simulink model "Long_Simul_1"  (R2022b)
settings: Solver=VariableStepAuto  StartTime=0.0  StopTime=Inf  RelTol=1e-3
values from neighbouring files (symbols this model uses):
  Af = 4    [Long_Simul_1_Initialize.m]    (also in Long_Simul_2_Initialize.m; Long_Simul_3_Initialize.m)
  Brake_Input_Amplitude = 100    [Long_Simul_1_Initialize.m]    (also in Long_Simul_2_Initialize.m = 10; Long_Simul_3_Initialize.m = 10)
  Brake_Input_start_time = 8    [Long_Simul_1_Initialize.m]    (also in Long_Simul_2_Initialize.m; Long_Simul_3_Initialize.m)
  C_long = 6*10^4    (= 60000)    [Long_Simul_1_Initialize.m]
  Cd = 0.3    [Long_Simul_1_Initialize.m]    (also in Long_Simul_2_Initialize.m; Long_Simul_3_Initialize.m)
  g = 9.81    [Long_Simul_1_Initialize.m]    (also in Long_Simul_2_Initialize.m; Long_Simul_3_Initialize.m)
  I_wheel = 0.8    [Long_Simul_1_Initialize.m]    (also in Long_Simul_2_Initialize.m; Long_Simul_3_Initialize.m)
  m = 1500    [Long_Simul_1_Initialize.m]    (also in Long_Simul_2_Initialize.m; Long_Simul_3_Initialize.m)
  r_eff = rw * sin(phi)/phi    [Long_Simul_1_Initialize.m]    (also in Long_Simul_2_Initialize.m; Long_Simul_3_Initialize.m)
  R_roll = 0.015    [Long_Simul_1_Initialize.m]    (also in Long_Simul_2_Initialize.m)
  rho = 1.225    [Long_Simul_1_Initialize.m]    (also in Long_Simul_2_Initialize.m; Long_Simul_3_Initialize.m)
  Throttle_Input_Amplitude = 30    [Long_Simul_1_Initialize.m]    (also in Long_Simul_2_Initialize.m; Long_Simul_3_Initialize.m = 50)
  Throttle_Input_period = 4    [Long_Simul_1_Initialize.m]    (also in Long_Simul_2_Initialize.m; Long_Simul_3_Initialize.m)
settings Model: Creator=lego0  LastModifiedBy=lego0

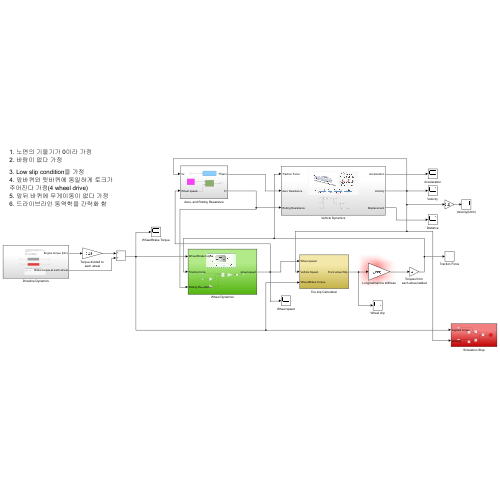
[thumbnail: Simulink's stored preview of the top-level diagram]
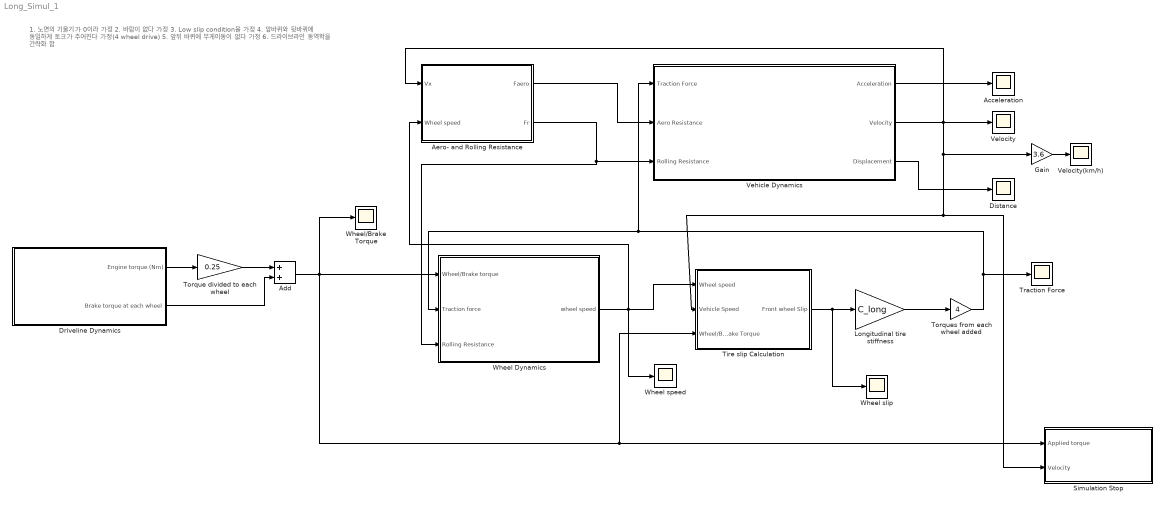
== system Long_Simul_1 ==
  note: 1. 노면의 기울기가 0이라 가정
      | 2. 바람이 없다 가정
      |
      | 3. Low slip condition을 가정
      | 4. 앞바퀴와 뒷바퀴에 동일하게 토크가 주어진다 가정(4 wheel drive)
      | 5. 앞뒤 바퀴에 무게이동이 없다 가정
      | 6. 드라이브라인 동역학을 간략화 함
  Acceleration : Scope
  Add : Sum
  Aero- and Rolling Resistance : Subsystem
  Distance : Scope
  Driveline Dynamics : Subsystem
  Gain : Gain  Gain=3.6
  Longitudinal tire stiffness : Gain  Gain=C_long
  Simulation Stop : Subsystem
  Tire slip Calculation : Subsystem
  Torque divided to each wheel : Gain  Gain=0.25
  Torques from each wheel added : Gain  Gain=4
  Traction Force : Scope
  Vehicle Dynamics : Subsystem
  Velocity : Scope
  Velocity(km/h) : Scope
  Wheel Dynamics : Subsystem
  Wheel slip : Scope
  Wheel speed : Scope
  Wheel/Brake Torque : Scope
  wires:
  Wheel Dynamics/1(wheel speed) -> Wheel speed/1, Aero- and Rolling Resistance/2(Wheel speed), Tire slip Calculation/1(Wheel speed)
  Tire slip Calculation/1(Front wheel Slip) -> Wheel slip/1, Longitudinal tire stiffness/1
  Longitudinal tire stiffness/1 -> Torques from each wheel added/1
  Vehicle Dynamics/1(Acceleration) -> Acceleration/1
  Vehicle Dynamics/2(Velocity) -> Tire slip Calculation/2(Vehicle Speed), Simulation Stop/2(Velocity), Gain/1, Velocity/1, Aero- and Rolling Resistance/1(Vx)
  Vehicle Dynamics/3(Displacement) -> Distance/1
  Gain/1 -> Velocity(km/h)/1
  Driveline Dynamics/2(Brake torque at each wheel) -> Add/2
  Aero- and Rolling Resistance/2(Fr) -> Wheel Dynamics/3(Rolling Resistance), Vehicle Dynamics/3(Rolling Resistance)
  Aero- and Rolling Resistance/1(Faero) -> Vehicle Dynamics/2(Aero Resistance)
  Add/1 -> Wheel Dynamics/1(Wheel/Brake torque), Tire slip Calculation/3(Wheel/Brake Torque), Simulation Stop/1(Applied torque), Wheel/Brake Torque/1
  Torques from each wheel added/1 -> Vehicle Dynamics/1(Traction Force), Wheel Dynamics/2(Traction force), Traction Force/1
  Driveline Dynamics/1(Engine torque (Nm)) -> Torque divided to each wheel/1
  Torque divided to each wheel/1 -> Add/1

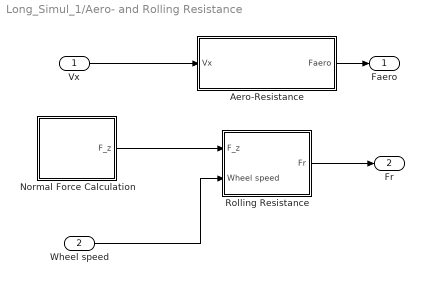
== system Long_Simul_1/Aero- and Rolling Resistance ==
  Vx : Inport
  Wheel speed : Inport  Port=2
  Aero-Resistance : Subsystem
  Normal Force Calculation : Subsystem
  Rolling Resistance : Subsystem
  Faero : Outport
  Fr : Outport  Port=2
  wires:
  Rolling Resistance/1(Fr) -> Fr/1
  Normal Force Calculation/1(F_z) -> Rolling Resistance/1(F_z)
  Vx/1 -> Aero-Resistance/1(Vx)
  Wheel speed/1 -> Rolling Resistance/2(Wheel speed)
  Aero-Resistance/1(Faero) -> Faero/1

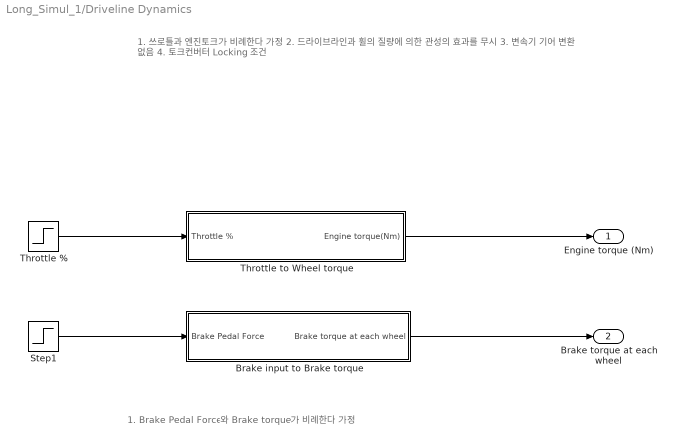
== system Long_Simul_1/Driveline Dynamics ==
  note: 1. 쓰로틀과 엔진토크가 비례한다 가정
      | 2. 드라이브라인과 휠의 질량에 의한 관성의 효과를 무시
      | 3. 변속기 기어 변환 없음
      | 4. 토크컨버터 Locking 조건
  note: 1. Brake Pedal Force와 Brake torque가 비례한다 가정
  Brake input to Brake torque : Subsystem
  Step1 : Step  Time=Brake_Input_start_time  After=Brake_Input_Amplitude  SampleTime=0
  Throttle % : Step  Time=Throttle_Input_period  Before=Throttle_Input_Amplitude  After=0  SampleTime=0
  Throttle to Wheel torque : Subsystem
  Engine torque (Nm) : Outport
  Brake torque at each wheel : Outport  Port=2
  wires:
  Throttle to Wheel torque/1(Engine torque(Nm)) -> Engine torque (Nm)/1
  Step1/1 -> Brake input to Brake torque/1(Brake Pedal Force)
  Throttle %/1 -> Throttle to Wheel torque/1(Throttle %)
  Brake input to Brake torque/1(Brake torque at each wheel) -> Brake torque at each wheel/1

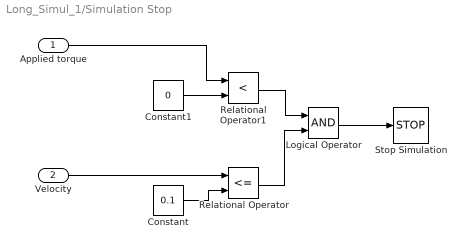
== system Long_Simul_1/Simulation Stop ==
  Applied torque : Inport
  Velocity : Inport  Port=2
  Constant : Constant  Value=0.1
  Constant1 : Constant  Value=0
  Logical Operator : Logic  AllPortsSameDT=off  OutDataTypeStr=boolean
  Relational Operator : RelationalOperator  Operator=<=  OutDataTypeStr=boolean  RndMeth=Simplest  InputSameDT=off
  Relational Operator1 : RelationalOperator  Operator=<  OutDataTypeStr=boolean  RndMeth=Simplest  InputSameDT=off
  Stop Simulation : Stop
  wires:
  Relational Operator1/1 -> Logical Operator/1
  Relational Operator/1 -> Logical Operator/2
  Constant/1 -> Relational Operator/2
  Constant1/1 -> Relational Operator1/2
  Logical Operator/1 -> Stop Simulation/1
  Velocity/1 -> Relational Operator/1
  Applied torque/1 -> Relational Operator1/1

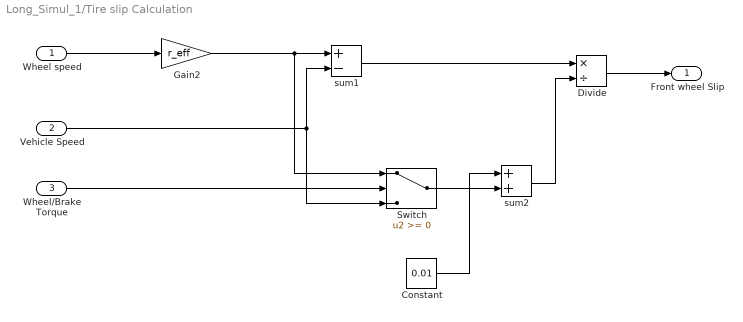
== system Long_Simul_1/Tire slip Calculation ==
  Wheel speed : Inport
  Vehicle Speed : Inport  Port=2
  Wheel/Brake Torque : Inport  Port=3
  Constant : Constant  Value=0.01
  Divide : Product  Inputs=*/
  Gain2 : Gain  Gain=r_eff
  Switch : Switch  SaturateOnIntegerOverflow=off  InputSameDT=off
  sum1 : Sum  Inputs=+-
  sum2 : Sum
  Front wheel Slip : Outport  VectorParamsAs1DForOutWhenUnconnected=off
  wires:
  Vehicle Speed/1 -> sum1/2, Switch/3
  Gain2/1 -> Switch/1, sum1/1
  Wheel speed/1 -> Gain2/1
  sum1/1 -> Divide/1
  Divide/1 -> Front wheel Slip/1
  Switch/1 -> sum2/2
  sum2/1 -> Divide/2
  Constant/1 -> sum2/1
  Wheel/Brake Torque/1 -> Switch/2

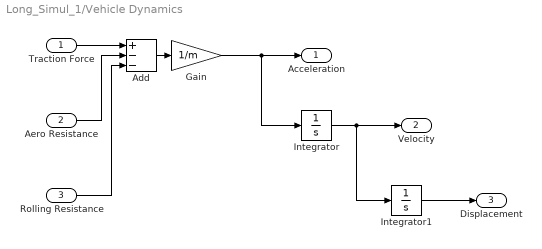
== system Long_Simul_1/Vehicle Dynamics ==
  Traction Force : Inport
  Aero Resistance : Inport  Port=2
  Rolling Resistance : Inport  Port=3
  Add : Sum  Inputs=+--
  Gain : Gain  Gain=1/m
  Integrator : Integrator
  Integrator1 : Integrator
  Acceleration : Outport
  Velocity : Outport  Port=2
  Displacement : Outport  Port=3
  wires:
  Integrator1/1 -> Displacement/1
  Gain/1 -> Integrator/1, Acceleration/1
  Integrator/1 -> Integrator1/1, Velocity/1
  Add/1 -> Gain/1
  Traction Force/1 -> Add/1
  Aero Resistance/1 -> Add/2
  Rolling Resistance/1 -> Add/3

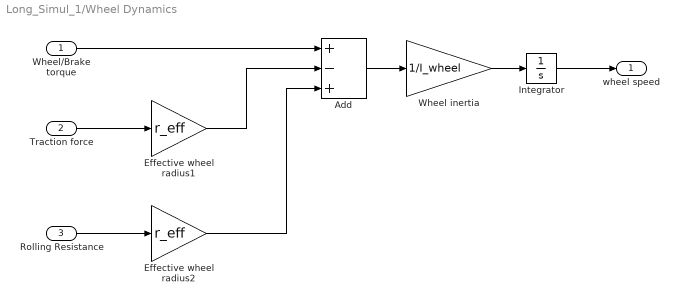
== system Long_Simul_1/Wheel Dynamics ==
  Wheel/Brake torque : Inport
  Traction force : Inport  Port=2
  Rolling Resistance : Inport  Port=3
  Add : Sum  Inputs=+-+
  Effective wheel radius1 : Gain  Gain=r_eff
  Effective wheel radius2 : Gain  Gain=r_eff
  Integrator : Integrator
  Wheel inertia : Gain  Gain=1/I_wheel
  wheel speed : Outport
  wires:
  Wheel inertia/1 -> Integrator/1
  Integrator/1 -> wheel speed/1
  Add/1 -> Wheel inertia/1
  Wheel/Brake torque/1 -> Add/1
  Traction force/1 -> Effective wheel radius1/1
  Rolling Resistance/1 -> Effective wheel radius2/1
  Effective wheel radius1/1 -> Add/2
  Effective wheel radius2/1 -> Add/3

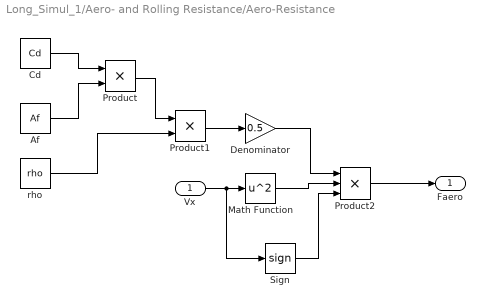
== system Long_Simul_1/Aero- and Rolling Resistance/Aero-Resistance ==
  Vx : Inport
  Af : Constant  Value=Af
  Cd : Constant  Value=Cd
  Denominator : Gain  Gain=0.5
  Math Function : Math  Operator=square  SignedPower=on
  Product : Product
  Product1 : Product
  Product2 : Product  Inputs=3
  Sign : Signum
  rho : Constant  Value=rho
  Faero : Outport  VectorParamsAs1DForOutWhenUnconnected=off
  wires:
  Af/1 -> Product/2
  Product1/1 -> Denominator/1
  Denominator/1 -> Product2/1
  Vx/1 -> Sign/1, Math Function/1
  rho/1 -> Product1/2
  Cd/1 -> Product/1
  Math Function/1 -> Product2/2
  Product/1 -> Product1/1
  Sign/1 -> Product2/3
  Product2/1 -> Faero/1

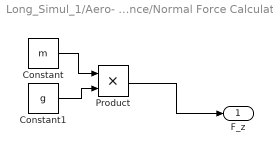
== system Long_Simul_1/Aero- and Rolling Resistance/Normal Force Calculation ==
  Constant : Constant  Value=m
  Constant1 : Constant  Value=g
  Product : Product
  F_z : Outport
  wires:
  Product/1 -> F_z/1
  Constant1/1 -> Product/2
  Constant/1 -> Product/1

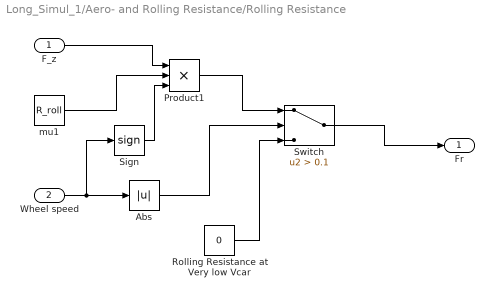
== system Long_Simul_1/Aero- and Rolling Resistance/Rolling Resistance ==
  F_z : Inport
  Wheel speed : Inport  Port=2
  Abs : Abs  SaturateOnIntegerOverflow=off
  Product1 : Product  Inputs=3
  Rolling Resistance at Very low Vcar : Constant  Value=0
  Sign : Signum
  Switch : Switch  Criteria=u2 > Threshold  Threshold=0.1  SaturateOnIntegerOverflow=off  InputSameDT=off
  mu1 : Constant  Value=R_roll
  Fr : Outport  VectorParamsAs1DForOutWhenUnconnected=off
  wires:
  F_z/1 -> Product1/1
  Product1/1 -> Switch/1
  Rolling Resistance at Very low Vcar/1 -> Switch/3
  mu1/1 -> Product1/2
  Wheel speed/1 -> Sign/1, Abs/1
  Abs/1 -> Switch/2
  Sign/1 -> Product1/3
  Switch/1 -> Fr/1

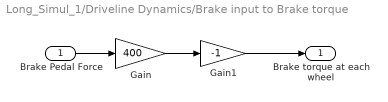
== system Long_Simul_1/Driveline Dynamics/Brake input to Brake torque ==
  Brake Pedal Force : Inport
  Gain : Gain  Gain=400
  Gain1 : Gain  Gain=-1
  Brake torque at each wheel : Outport  VectorParamsAs1DForOutWhenUnconnected=off
  wires:
  Gain/1 -> Gain1/1
  Brake Pedal Force/1 -> Gain/1
  Gain1/1 -> Brake torque at each wheel/1

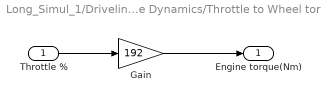
== system Long_Simul_1/Driveline Dynamics/Throttle to Wheel torque ==
  Throttle % : Inport
  Gain : Gain  Gain=192
  Engine torque(Nm) : Outport  VectorParamsAs1DForOutWhenUnconnected=off
  wires:
  Throttle %/1 -> Gain/1
  Gain/1 -> Engine torque(Nm)/1
